simulink model "FMS"  (R2018b)
settings: configuration reference "fms_config" (kept outside this file)
values from neighbouring files (symbols this model uses):
  FMS_EXPORT = Simulink.Parameter(FMS_EXPORT_VALUE)    [fms_model_init.m]
  FMS_PARAM = Simulink.Parameter(FMS_PARAM_VALUE)    [fms_model_init.m]
undefined symbols (not defined in the file or in its folder): actuator_cmd, ay_cmd, cmd_mask, ControlMode, ctrl_mode, DiscIntNeverNeededParam, FMS_Cmd, mode, PilotMode, r_cmd, reset, state, status, theta_cmd, timestamp, u_cmd, VehicleState, VehicleStatus, w_cmd, wp_consume, wp_current
libraries: simulink x27, FMT_Model_Lib x21, hdlsllib x4
(part 3 of 3)

== stateflow chart FMS/FMS State Machine ==
  state Command_Listener [parallel]
    settings: executionOrder=1
    state Send
      entry:
      % Send command
      M.data=save_cmd;
      send(M);
    state Listen
    state Check
      entry:
      valid_cmd = CheckCmdValid(save_cmd, mode, INS_Out.flag);
    (default) -> Listen
    Send -> Listen
    Listen -> Check : [hasChanged(cmd) && ...
        | cmd ~= FMS_Cmd.None]{save_cmd = cmd;}
    Check -> Listen [order 2]
    Check -> Send [order 1] : [valid_cmd == true]
  state Vehicle [parallel]
    du:
    % if mission data updated, reset waypoint index
    if hasChanged(mission_timestamp)
    wp_consume = 0;
    wp_index = 1;
    end
    settings: executionOrder=3
    state moved = StickMoved(stick_val,pilot_cmd) [function]
    state Arm
      en:
      status = VehicleStatus.Arm;
      state SubMode
        en:
        stick_val = [Pilot_Cmd.stick_yaw; Pilot_Cmd.stick_throttle; Pilot_Cmd.stick_roll; Pilot_Cmd.stick_pitch];
        state Hold
          en:
          state = VehicleState.Hold;
        state Return
          en:
          state = VehicleState.Return;
        SubMode -> Hold [order 1] : M[M.data==FMS_Cmd.Pause]
      state Auto
        state Offboard
          en:
          Cmd_In.offboard_psi_0 = INS_Out.psi;
          state Loiter
            en:
            state = VehicleState.Hold;
          state Run
            en:
            state = VehicleState.Offboard;
          (default) -> (junction 955)
          (junction 955) -> Vehicle.Arm.Auto.Offboard.Loiter [order 2]
          (junction 955) -> Run [order 1] : [auto_cmd_valid == 1]
          Run -> Vehicle.Arm.Auto.Offboard.Loiter : [auto_cmd_valid == 0]
          Vehicle.Arm.Auto.Offboard.Loiter -> Run : [auto_cmd_valid == 1]
        state Mission
          en:
          % Reference location of latitude and longitude, specified as an m-by-2 array, in degrees
          llo = [INS_Out.lat, INS_Out.lon] * (180/pi);
          Cmd_In.cur_waypoint =[INS_Out.x_R; INS_Out.y_R; INS_Out.h_R];
          state pos = LLA2FLAT(lla,llo,href,psio) [function]
          state Loiter
            en:
            state = VehicleState.Hold;
          state NextWP
            en:
            if wp_index <= Mission_Data.valid_items
            nav_cmd = Mission_Data.command(wp_index);
            else
            nav_cmd = uint16(NAV_Cmd.None);
            % updated consumed waypoints
            wp_consume = wp_index - 1;
            end
          state Waypoint
            en:
            % Geodetic coordinates (latitude, longitude, and altitude), specified as an m-by-3 array in [degrees degrees meters]
            % Altitude add home(3) here because the altitude when takeoff could be non-zero
            lla = [double(Mission_Data.x(wp_index))*1e-7, double(Mission_Data.y(wp_index))*1e-7, double(-(Mission_Data.z(wp_index)))];
            % target waypoint
            Cmd_In.sp_waypoint = LLA2FLAT(lla, llo, 0, 0) + home;
            state = VehicleState.Mission;
          state Return
            en:
            Cmd_In.cur_waypoint = Cmd_In.sp_waypoint;
            Cmd_In.sp_waypoint = [home(1); home(2); INS_Out.h_R];
            state = VehicleState.Return;
          Mission -> NextWP : [hasChanged(mission_timestamp)]
          (junction 908) -> (junction 910) : {wp_index = wp_index + 1;}
          (junction 910) -> NextWP
          (junction 873) -> (junction 908)
          (default) -> NextWP
          (junction 917) -> Vehicle.Arm.Auto.Mission.Loiter
          (junction 879) -> (junction 873)
          NextWP -> (junction 917) [order 3]
          NextWP -> Waypoint [order 1] : [nav_cmd == NAV_Cmd.Waypoint]
          Waypoint -> (junction 879) : [norm([INS_Out.x_R;INS_Out.y_R]-Cmd_In.sp_waypoint(1:2)) <= accept_radius]
              | {Cmd_In.cur_waypoint = Cmd_In.sp_waypoint;}
          (junction 915) -> (junction 879)
          NextWP -> Vehicle.Arm.Auto.Mission.Return [order 2] : [nav_cmd == NAV_Cmd.Return]
          Vehicle.Arm.Auto.Mission.Return -> (junction 915) : [norm([INS_Out.x_R; INS_Out.y_R]-Cmd_In.sp_waypoint(1:2)) < 0.5]
        state InvalidAutoMode
        (default) -> (junction 43)
        (junction 43) -> Offboard [order 1] : [mode == PilotMode.Offboard]
        (junction 43) -> (junction 134) [order 2]
        (junction 134) -> Mission [order 1] : [mode == PilotMode.Mission]
        (junction 134) -> InvalidAutoMode [order 2]
        InvalidAutoMode -> (junction 370)
      state Assist
        state InvalidAssistMode
        state Stabilize
          en:
          state = VehicleState.Stabilize;
        state Altitude
          en:
          state = VehicleState.Altitude;
        state Position
          en:
          state = VehicleState.Position;
        (default) -> (junction 190)
        (junction 190) -> (junction 949) [order 2]
        (junction 949) -> (junction 196) [order 2]
        (junction 196) -> InvalidAssistMode [order 2]
        (junction 190) -> Stabilize [order 1] : [mode == PilotMode.Stabilize]
        (junction 949) -> Altitude [order 1] : [mode == PilotMode.Altitude]
        (junction 196) -> Position [order 1] : [mode == PilotMode.Position]
      state Manual
        state InValidManualMode
        state Manual
          en:
          state = VehicleState.Manual;
        (default) -> (junction 410)
        (junction 410) -> InValidManualMode [order 2]
        (junction 410) -> Vehicle.Arm.Manual.Manual [order 1] : [mode == PilotMode.Manual]
      state InvalidArmMode
      Vehicle.Arm -> Vehicle.Arm.SubMode.Return [order 2] : M[M.data==FMS_Cmd.Return]
          | {Cmd_In.sp_waypoint = [home(1); home(2); INS_Out.h_R]}
      Hold -> Vehicle.Arm : M[M.data==FMS_Cmd.Continue ...
          | && mode ~= PilotMode.None]
      Auto -> Hold : M[M.data==FMS_Cmd.Pause]
      SubMode -> (junction 117) [order 1] : [StickMoved(stick_val, Pilot_Cmd) && ...
          | mode ~= PilotMode.None]
      Vehicle.Arm -> (junction 117) [order 1] : [hasChanged(mode) && ...
          | mode ~= PilotMode.None]
      (junction 117) -> Auto [order 1] : [getArmMode(mode) == 3]
      (default) -> (junction 117)
      (junction 117) -> (junction 140) [order 2]
      (junction 140) -> Assist [order 1] : [getArmMode(mode)  == 2]
      (junction 140) -> (junction 240) [order 2]
      (junction 240) -> Vehicle.Arm.Manual [order 1] : [getArmMode(mode)  == 1]
      (junction 240) -> InvalidArmMode [order 2]
    state Standby
      en:
      % check if mission takeoff is valid
      if mode==PilotMode.Mission
      if wp_index <= Mission_Data.valid_items > 0
      % set mission takeoff flag, so enter mission mode after 2s
      prep_mission = 1;
      else
      send(DisarmEvent);
      end
      end
      % set current position as home
      home = [INS_Out.x_R; INS_Out.y_R; INS_Out.h_R];
      % enter standby state
      state = VehicleState.Standby;
      status = VehicleStatus.Standby;
      ex:
      % on exit, unset flag
      prep_mission = 0;
    state Disarm
      en:
      state = VehicleState.Disarm;
      status = VehicleStatus.Disarm;
    InValidManualMode -> Vehicle
    Vehicle.Arm.SubMode.Return -> (junction 330) : [norm([INS_Out.x_R,INS_Out.y_R]-[home(1),home(2)]) ...
        | <= accept_radius]
    (junction 330) -> Vehicle.Disarm
    InvalidAssistMode -> Vehicle
    (junction 370) -> Vehicle
    (default) -> Vehicle.Disarm
    Standby -> Vehicle.Disarm [order 2] : after(10, sec) || DisarmEvent
    Standby -> Vehicle.Arm [order 1] : [ManualArmEvent(Pilot_Cmd) == 1 &&...
        | mode ~= PilotMode.None]
    Vehicle.Disarm -> Standby : M[M.data==FMS_Cmd.PreArm]
    Standby -> Vehicle.Arm [order 4] : [mode == PilotMode.Offboard && ...
        | auto_cmd_valid]
    Vehicle -> Vehicle.Disarm : M[M.data==FMS_Cmd.Disarm]
    Standby -> (junction 903) [order 3] : [duration(prep_mission == 1) >= 2]
    (junction 903) -> Vehicle.Arm
    InvalidArmMode -> Vehicle
  state Combo_Stick [parallel]
    settings: executionOrder=2
    state res = BottomRight(pilot_cmd) [function]
      (default) -> (junction 285) : {res = (pilot_cmd.stick_throttle < -0.8) && ...
          | (pilot_cmd.stick_yaw > 0.8);}
    state Idle
      du:
      bl = BottomLeft(Pilot_Cmd);
      br = BottomRight(Pilot_Cmd);
    state Arm
      en:
      M.data=FMS_Cmd.PreArm;
      send(M);
    state res = BottomLeft(pilot_cmd) [function]
      (default) -> (junction 298) : {res = (pilot_cmd.stick_throttle < -0.8) && ...
          | (pilot_cmd.stick_yaw < -0.8);}
    state Disarm
      en:
      send(DisarmEvent, Vehicle)
    (default) -> Idle
    Combo_Stick.Arm -> Idle : [~BottomRight(Pilot_Cmd)]
    Idle -> Combo_Stick.Arm [order 1] : [duration(br)>1.5]
    Idle -> Combo_Stick.Disarm [order 2] : [duration(bl)>1.5]
    Combo_Stick.Disarm -> Idle : [~BottomLeft(Pilot_Cmd)]
  data: cmd_in function_input; mode_in function_input; valid function_output; ins_flag function_input; pilotMode function_input; armMode function_output; pilot_cmd function_input; trigger function_output; stick_val function_input double size=4; moved function_output; pilot_cmd function_input Bus: Pilot_Cmd_Bus size=1; lla function_input double size=[1 3]; llo function_input double size=[1 2]; href function_input double size=1; pos function_output; psio function_input double size=1; res function_output; pilot_cmd function_input; res function_output; pilot_cmd function_input; state output Enum: VehicleState; cmd input; valid_cmd local; M local Enum: FMS_Cmd; mode input; Pilot_Cmd input Bus: Pilot_Cmd_Bus; INS_Out input Bus: INS_Out_Bus; Mission_Data input Bus: Mission_Data_Bus; home local; stick_val local; bl local =false; br local =false; nav_cmd local uint16; wp_consume output uint8 =uint8(0); wp_index output uint8 =uint8(1); Cmd_In output Bus: Commander_In_Bus; mission_timestamp input uint32 =uint32(0); status local Enum: VehicleStatus =VehicleStatus.None; llo local; lla local; save_cmd local Enum: FMS_Cmd; accept_radius input; prep_mission local =0; auto_cmd_valid input
  events: DisarmEvent local FUNCTION_CALL_EVENT
  function valid = CheckCmdValid(cmd_in, mode_in, ins_flag):
    | function valid = CheckCmdValid(cmd_in, mode_in, ins_flag)
    | 
    | % bit1 |    bit2    |    bit3  |   bit4  | bit5  | bit6  |bit7|bit8|bit9
    | % init | standstill | attitude | heading | speed | LLA   | xy | h | h_AGL
    | 
    | valid = false;
    | 
    | % TODO: Add more checks
    | switch cmd_in
    |     case {FMS_Cmd.Takeoff, FMS_Cmd.Land, FMS_Cmd.Return, FMS_Cmd.Pause}
    |         if ~bitget(ins_flag, 1) || ~bitget(ins_flag, 3) || ~bitget(ins_flag, 4)
    |             valid = true;
    |         end
    |         % these modes need position valid
    |         if bitget(ins_flag, 5) && bitget(ins_flag, 7) && bitget(ins_flag, 8)
    |             valid = true;
    |         end
    |     case FMS_Cmd.PreArm
    |         if ~bitget(ins_flag, 1) || ~bitget(ins_flag, 3) || ~bitget(ins_flag, 4)
    |             return;
    |         end
    |         
    |         switch mode_in
    |             case {PilotMode.Position, PilotMode.Mission, PilotMode.Offboard}
    |                 if bitget(ins_flag, 5) && bitget(ins_flag, 7) && bitget(ins_flag, 8)
    |                     valid = true;
    |                 end
    |             case PilotMode.Altitude
    |                 if bitget(ins_flag, 8)
    |                     valid = true;
    |                 end
    |             case PilotMode.Stabilize
    |                 valid = true;
    |             otherwise
    |                 % do nothing
    |         end
    |     case FMS_Cmd.Continue
    |         if mode_in == PilotMode.Offboard || mode_in == PilotMode.Mission
    |            valid = true; 
    |         end
    |     case FMS_Cmd.Disarm
    |         valid = true;   % always allowed disarm
    |     otherwise
    |         % do nothing
    | end
    | 
    | return;
  function armMode = getArmMode(pilotMode):
    | function armMode = getArmMode(pilotMode)
    | 
    | % Map pilot mode to arm mode
    | switch pilotMode
    |     case PilotMode.Manual
    |         armMode = 1;    % manual
    |     case {PilotMode.Acro, PilotMode.Stabilize, PilotMode.Altitude, PilotMode.Position}
    |         armMode = 2;    % asist
    |     case {PilotMode.Mission, PilotMode.Offboard}
    |         armMode = 3;    % auto
    |     otherwise
    |         armMode = 0;    % unknown
    | end
    | 
    | end
  function trigger = ManualArmEvent(pilot_cmd):
    | function trigger = ManualArmEvent(pilot_cmd)
    | 
    | trigger = 0;
    | 
    | % Map pilot mode to arm mode
    | switch pilot_cmd.mode
    |     case {PilotMode.Stabilize, PilotMode.Altitude, PilotMode.Position}
    |         if pilot_cmd.stick_throttle > 0
    |             trigger = 1;
    |         end
    |     otherwise
    |         % do nothing
    | end
    | 
    | end

== stateflow chart FMS/FMS Commander/Commander/Arm/Assist/Position/Speed Command/Detect Movement/Motion State ==
  state Hold
    entry:
    state=MotionState.Hold;
  state Move
    entry:
    state=MotionState.Move;
  state Brake
    entry:
    state=MotionState.Brake;
  (default) -> Move
  Hold -> Move : [motion_req==1]
  Move -> Brake : [motion_req==0]
  Brake -> Move [order 2] : [motion_req==1]
  Brake -> Hold [order 1] : [speed<=0.1 || after(2.0, sec)]
  data: state output Enum: MotionState; motion_req input; speed input

== stateflow chart FMS/FMS Commander/Commander/Arm/Assist/Altitude/Altitude Command/Detect Movement/Motion Status ==
  state Hold
    entry:
    state=MotionState.Hold;
  state Move
    entry:
    state=MotionState.Move;
  state Brake
    entry:
    state=MotionState.Brake;
  (default) -> Move
  Hold -> Move : [motion_req==1]
  Move -> Brake : [motion_req==0]
  Brake -> Move [order 2] : [motion_req==1]
  Brake -> Hold [order 1] : [speed<=0.1 || after(1.5, sec)]
  data: state output Enum: MotionState; motion_req input; speed input
